simulink model "ZT_VehCtrl_18B_CAN"  (R2018b)
settings: Solver=FixedStepAuto  StartTime=0.0  StopTime=inf  FixedStep=0.005  RelTol=1e-3
InitFcn:
  | mbd_mpc_consistency_checks(bdroot(gcs));
values from neighbouring files (symbols this model uses):
  BatoverTempTh = single(80)    [VCU_INIT.m]
  BRS_PwrValid = single(5)    [VCU_INIT.m]
  BRSEnSpdTh1 = single(10)    [VCU_INIT.m]
  BRSEnSpdTh2 = single(20)    [VCU_INIT.m]
  MCUTempAlarmTh = single (60)    [VCU_INIT.m]
  mps2kmh = single(3.6)    [VCU_INIT.m]
  MtrPwrFac = single(1/9550)    [VCU_INIT.m]
  MtrTempAlarmTh = single (50)    [VCU_INIT.m]
  Padle1Signal1_Th = [PadleSignal1_min,PadleSignal1_max]    [VCU_INIT.m]
  Padle1Signal2_Th = [PadleSignal2_min,PadleSignal2_max]    [VCU_INIT.m]
  PadleSignal1_max = 3.84    [VCU_INIT.m]
  PadleSignal1_min = 0.75    [VCU_INIT.m]
  PadleSignal2_max = 1.92    [VCU_INIT.m]
  PadleSignal2_min = 0.375    [VCU_INIT.m]
  PadleValid = 0.05    [VCU_INIT.m]
  PwrLimFactor = single(0.5)    [VCU_INIT.m]
  Ratio = single(1)    [VCU_INIT.m]
  rpm2mps = single(2*pi/60 * WhlRadius/Ratio)    [VCU_INIT.m]
  SOCLowTh = single(20)    [VCU_INIT.m]
  VehPwrBackwardMax = VehPwrMax * single(0.3)    [VCU_INIT.m]
  VehPwrMax = single(MtrPwrMax * 4)    [VCU_INIT.m]
  VehTrqBackwardMax = VehTrqMax * single(0.3)    [VCU_INIT.m]
  VehTrqMax = single(MtrTrqMax * Ratio *4)    [VCU_INIT.m]
  WhlRadius = single(1)    [VCU_INIT.m]
undefined symbols (not defined in the file or in its folder): Delay_Charge, Delay_Discharge, fifo_0_vect, fifo_1_vect, LQFP, pts1_fifo_0_vect, pts1_fifo_1_vect, pts2_fifo_0_vect, pts2_fifo_1_vect, pts3_fifo_0_vect, pts3_fifo_1_vect, pts4_fifo_0_vect, pts4_fifo_1_vect
libraries: mbd_mpc574x_ec_toolbox x157, canmsglib x74, simulink x38
(part 11 of 12)

== system ZT_VehCtrl_18B_CAN/SigIn/CAN1/TM MCU STATUS 1/UNPACK ==
  ID : Inport
  data : Inport  Port=2
  length : Inport  Port=3
  timestamp : Inport  Port=4
  Action Port : ActionPort  ActionType=case
  Add : Sum
  Bus Creator : BusCreator  Inputs=7  OutDataTypeStr=Bus: CAN_MESSAGE_BUS  NonVirtualBus=on
  Bus Creator1 : BusCreator  Inputs=7
  CAN Unpack6 : canmsglib/CAN Unpack  CANdbFile=D:\VCU\VCU_SL_ZhengZhou\ZT2\模型与接口\CAN_DBC\动力CANB_GBK.dbc  MsgList=(none)  MsgName=TM_MCU_STATUS_1  MsgIDType=Extended (29-bit identifier)  MsgIdentifier=218038277  MsgLength=8  SignalInfo=Active_Discharge_Enable_Feedback$53$1$1$2$1$0$1$0$-Inf$Inf$#IGBT_Enable_Feedback$54$1$1$2$1$0$1$0$-Inf$Inf$#Life_counter$60$4$1$2$1$0$1$0$-Inf$Inf$#Motor_AC_Current$32$16$1$2$1$0$1.000000e-01$0$0$1000$#Motor_Speed$0$16$1$2$1$0$1$-15000$-15000$15000$#Motor_Torque$16$16$1$2$1$0$1$-5000$-5000$5000$#Precharge_Allow$52$1$1$2$1$0$1$0$-Inf$Inf$#  NSignals=7  IDPort=off  TimestampPort=off  ErrorPort=off  RemotePort=off  LengthPort=off  StatusPort=off  StartBits=str2num('[int32(53);int32(54);int32(60);int32(32);int32(0);int32(16);int32(52)]')  SignalSizes=str2num('[int32(1);int32(1);int32(4);int32(16);int32(16);int32(16);int32(1)]')  ByteOrders=str2num('[int32(1);int32(1);int32(1);int32(1);int32(1);int32(1);int32(1)]')  DataTypes=str2num('[int32(2);int32(2);int32(2);int32(2);int32(2);int32(2);int32(2)]')  MultiplexTypes=str2num('[int32(1);int32(1);int32(1);int32(1);int32(1);int32(1);int32(1)]')  MultiplexValues=str2num('[double(0);double(0);double(0);double(0);double(0);double(0);double(0)]')  Factors=str2num('[double(1);double(1);double(1);double(1.000000e-01);double(1);double(1);double(1)]')  Offsets=str2num('[double(0);double(0);double(0);double(0);double(-15000);double(-5000);double(0)]')  Minimums=str2num('[double(-Inf);double(-Inf);double(-Inf);double(0);double(-15000);double(-5000);double(-Inf)]')  Maximums=str2num('[double(Inf);double(Inf);double(Inf);double(1000);double(15000);double(5000);double(Inf)]')  ApplyMinMax=off
      settings: SourceProductName=Simulink Real-Time  SourceProductBaseCode=XP  DataFormat=CANdb specified signals
  Constant : Constant  OutDataTypeStr=uint8
  Constant1 : Constant  OutDataTypeStr=uint8
  Constant4 : Constant  Value=0  OutDataTypeStr=uint8
  Constant5 : Constant  Value=0  OutDataTypeStr=uint8
  Data Store Read : DataStoreRead  DataStoreName=Cnt_TW1
  Data Store Write : DataStoreWrite  DataStoreName=Cnt_TW1
  Data Type Conversion{,14..15,17} (4 alike) : DataTypeConversion  OutDataTypeStr=uint8
  Data Type Conversion1 : DataTypeConversion  OutDataTypeStr=boolean
  Data Type Conversion18 : DataTypeConversion  OutDataTypeStr=uint32
  Data Type Conversion19 : DataTypeConversion  OutDataTypeStr=double
  Data Type Conversion2 : DataTypeConversion  OutDataTypeStr=boolean
  Data Type Conversion{3..6} (4 alike) : DataTypeConversion  OutDataTypeStr=single
  Data Type Conversion7 : DataTypeConversion  OutDataTypeStr=boolean
  Message : Outport
  wires:
  Bus Creator1/1 -> Message/1
  Data Type Conversion15/1 -> Bus Creator/3  "Remote"
  Data Type Conversion14/1 -> Bus Creator/2  "Length"
  Data Type Conversion/1 -> Bus Creator/1  "Extended"
  Bus Creator/1 -> CAN Unpack6/1  "CAN_Msg_In"
  Data Type Conversion17/1 -> Bus Creator/4  "Error"
  timestamp/1 -> Data Type Conversion19/1
  Data Type Conversion19/1 -> Bus Creator/6  "Timestamp"
  ID/1 -> Data Type Conversion18/1
  Constant5/1 -> Data Type Conversion17/1
  Constant1/1 -> Data Type Conversion/1
  Data Type Conversion18/1 -> Bus Creator/5  "ID"
  data/1 -> Bus Creator/7  "Data"
  length/1 -> Data Type Conversion14/1
  Constant4/1 -> Data Type Conversion15/1
  CAN Unpack6/1 -> Data Type Conversion1/1
  CAN Unpack6/2 -> Data Type Conversion2/1
  CAN Unpack6/3 -> Data Type Conversion3/1
  CAN Unpack6/4 -> Data Type Conversion4/1
  CAN Unpack6/5 -> Data Type Conversion5/1
  CAN Unpack6/6 -> Data Type Conversion6/1
  CAN Unpack6/7 -> Data Type Conversion7/1
  Data Type Conversion1/1 -> Bus Creator1/1  "Active_Discharge_Enable_Feedback"
  Data Type Conversion2/1 -> Bus Creator1/2  "IGBT_Enable_Feedback"
  Data Type Conversion3/1 -> Bus Creator1/3  "Life_counter"
  Data Type Conversion4/1 -> Bus Creator1/4  "Motor_AC_Current"
  Data Type Conversion5/1 -> Bus Creator1/5  "Motor_Speed"
  Data Type Conversion6/1 -> Bus Creator1/6  "Motor_Torque"
  Data Type Conversion7/1 -> Bus Creator1/7  "Precharge_Allow"
  Constant/1 -> Add/2
  Data Store Read/1 -> Add/1
  Add/1 -> Data Store Write/1

== system ZT_VehCtrl_18B_CAN/SigIn/CAN1/TM MCU STATUS 2/UNPACK ==
  ID : Inport
  data : Inport  Port=2
  length : Inport  Port=3
  timestamp : Inport  Port=4
  Action Port : ActionPort  ActionType=case
  Add : Sum
  Bus Creator : BusCreator  Inputs=7  OutDataTypeStr=Bus: CAN_MESSAGE_BUS  NonVirtualBus=on
  Bus Creator1 : BusCreator  Inputs=6
  CAN Unpack6 : canmsglib/CAN Unpack  CANdbFile=D:\VCU\VCU_SL_ZhengZhou\ZT2\Module\CAN_DBC\动力CANB_GBK.dbc  MsgList=(none)  MsgName=TM_MCU_STATUS2  MsgIDType=Extended (29-bit identifier)  MsgIdentifier=218038533  MsgLength=8  SignalInfo=Fail_Grade$48$4$1$2$1$0$1$0$-Inf$Inf$#Life_counter$60$4$1$2$1$0$1$0$-Inf$Inf$#MCU_temperature$8$8$1$2$1$0$1$-40$-40$215$#Motor_Temperature$0$8$1$2$1$0$1$-40$-40$215$#Torque_Limit_High$16$16$1$2$1$0$1$0$0$5000$#Torque_Limit_Low$32$16$1$2$1$0$1$-5000$-5000$0$#  NSignals=6  IDPort=off  TimestampPort=off  ErrorPort=off  RemotePort=off  LengthPort=off  StatusPort=off  StartBits=str2num('[int32(48);int32(60);int32(8);int32(0);int32(16);int32(32)]')  SignalSizes=str2num('[int32(4);int32(4);int32(8);int32(8);int32(16);int32(16)]')  ByteOrders=str2num('[int32(1);int32(1);int32(1);int32(1);int32(1);int32(1)]')  DataTypes=str2num('[int32(2);int32(2);int32(2);int32(2);int32(2);int32(2)]')  MultiplexTypes=str2num('[int32(1);int32(1);int32(1);int32(1);int32(1);int32(1)]')  MultiplexValues=str2num('[double(0);double(0);double(0);double(0);double(0);double(0)]')  Factors=str2num('[double(1);double(1);double(1);double(1);double(1);double(1)]')  Offsets=str2num('[double(0);double(0);double(-40);double(-40);double(0);double(-5000)]')  Minimums=str2num('[double(-Inf);double(-Inf);double(-40);double(-40);double(0);double(-5000)]')  Maximums=str2num('[double(Inf);double(Inf);double(215);double(215);double(5000);double(0)]')  ApplyMinMax=off
      settings: SourceProductName=Simulink Real-Time  SourceProductBaseCode=XP  DataFormat=CANdb specified signals
  Constant : Constant  OutDataTypeStr=uint8
  Constant1 : Constant  OutDataTypeStr=uint8
  Constant4 : Constant  Value=0  OutDataTypeStr=uint8
  Constant5 : Constant  Value=0  OutDataTypeStr=uint8
  Data Store Read : DataStoreRead  DataStoreName=Cnt_TW2
  Data Store Write : DataStoreWrite  DataStoreName=Cnt_TW2
  Data Type Conversion{,14..15,17} (4 alike) : DataTypeConversion  OutDataTypeStr=uint8
  Data Type Conversion{1..6} (6 alike) : DataTypeConversion  OutDataTypeStr=single
  Data Type Conversion18 : DataTypeConversion  OutDataTypeStr=uint32
  Data Type Conversion19 : DataTypeConversion  OutDataTypeStr=double
  Message : Outport
  wires:
  Constant4/1 -> Data Type Conversion15/1
  length/1 -> Data Type Conversion14/1
  data/1 -> Bus Creator/7  "Data"
  Data Type Conversion18/1 -> Bus Creator/5  "ID"
  Constant1/1 -> Data Type Conversion/1
  Constant5/1 -> Data Type Conversion17/1
  ID/1 -> Data Type Conversion18/1
  Data Type Conversion19/1 -> Bus Creator/6  "Timestamp"
  timestamp/1 -> Data Type Conversion19/1
  Data Type Conversion17/1 -> Bus Creator/4  "Error"
  Bus Creator/1 -> CAN Unpack6/1  "CAN_Msg_In"
  Data Type Conversion/1 -> Bus Creator/1  "Extended"
  Data Type Conversion14/1 -> Bus Creator/2  "Length"
  Data Type Conversion15/1 -> Bus Creator/3  "Remote"
  Bus Creator1/1 -> Message/1
  CAN Unpack6/4 -> Data Type Conversion4/1
  CAN Unpack6/3 -> Data Type Conversion3/1
  CAN Unpack6/5 -> Data Type Conversion5/1
  CAN Unpack6/2 -> Data Type Conversion2/1
  CAN Unpack6/6 -> Data Type Conversion6/1
  CAN Unpack6/1 -> Data Type Conversion1/1
  Data Type Conversion1/1 -> Bus Creator1/1  "Fail_Grade"
  Data Type Conversion2/1 -> Bus Creator1/2  "Life_counter"
  Data Type Conversion3/1 -> Bus Creator1/3  "MCU_temperature"
  Data Type Conversion4/1 -> Bus Creator1/4  "Motor_Temperature"
  Data Type Conversion5/1 -> Bus Creator1/5  "Torque_Limit_High"
  Data Type Conversion6/1 -> Bus Creator1/6  "Torque_Limit_Low"
  Constant/1 -> Add/2
  Add/1 -> Data Store Write/1
  Data Store Read/1 -> Add/1

== system ZT_VehCtrl_18B_CAN/SigIn/CAN1/TM MCU STATUS 3/UNPACK ==
  ID : Inport
  data : Inport  Port=2
  length : Inport  Port=3
  timestamp : Inport  Port=4
  Action Port : ActionPort  ActionType=case
  Add : Sum
  Bus Creator : BusCreator  Inputs=7  OutDataTypeStr=Bus: CAN_MESSAGE_BUS  NonVirtualBus=on
  Bus Creator1 : BusCreator  Inputs=5
  CAN Unpack6 : canmsglib/CAN Unpack  CANdbFile=D:\VCU\VCU_SL_ZhengZhou\ZT2\Module\CAN_DBC\动力CANB_GBK.dbc  MsgList=(none)  MsgName=TM_MCU_STATUS3  MsgIDType=Extended (29-bit identifier)  MsgIdentifier=218038789  MsgLength=8  SignalInfo=Alarm_Code$8$8$1$2$1$0$1$0$0$255$#DC_Current_A$16$16$1$2$1$0$1$-1000$-1000$1000$#DC_Voltage_V$32$16$1$2$1$0$1.000000e-01$0$0$1000$#Fault_Code$0$8$1$2$1$0$1$0$0$255$#Life_counter$48$4$1$2$1$0$1$0$0$15$#  NSignals=5  IDPort=off  TimestampPort=off  ErrorPort=off  RemotePort=off  LengthPort=off  StatusPort=off  StartBits=str2num('[int32(8);int32(16);int32(32);int32(0);int32(48)]')  SignalSizes=str2num('[int32(8);int32(16);int32(16);int32(8);int32(4)]')  ByteOrders=str2num('[int32(1);int32(1);int32(1);int32(1);int32(1)]')  DataTypes=str2num('[int32(2);int32(2);int32(2);int32(2);int32(2)]')  MultiplexTypes=str2num('[int32(1);int32(1);int32(1);int32(1);int32(1)]')  MultiplexValues=str2num('[double(0);double(0);double(0);double(0);double(0)]')  Factors=str2num('[double(1);double(1);double(1.000000e-01);double(1);double(1)]')  Offsets=str2num('[double(0);double(-1000);double(0);double(0);double(0)]')  Minimums=str2num('[double(0);double(-1000);double(0);double(0);double(0)]')  Maximums=str2num('[double(255);double(1000);double(1000);double(255);double(15)]')  ApplyMinMax=off
      settings: SourceProductName=Simulink Real-Time  SourceProductBaseCode=XP  DataFormat=CANdb specified signals
  Constant : Constant  OutDataTypeStr=uint8
  Constant1 : Constant  OutDataTypeStr=uint8
  Constant4 : Constant  Value=0  OutDataTypeStr=uint8
  Constant5 : Constant  Value=0  OutDataTypeStr=uint8
  Data Store Read : DataStoreRead  DataStoreName=Cnt_TW3
  Data Store Write : DataStoreWrite  DataStoreName=Cnt_TW3
  Data Type Conversion{,14..15,17} (4 alike) : DataTypeConversion  OutDataTypeStr=uint8
  Data Type Conversion{1..5} (5 alike) : DataTypeConversion  OutDataTypeStr=single
  Data Type Conversion18 : DataTypeConversion  OutDataTypeStr=uint32
  Data Type Conversion19 : DataTypeConversion  OutDataTypeStr=double
  Message : Outport
  wires:
  Bus Creator1/1 -> Message/1
  Data Type Conversion15/1 -> Bus Creator/3  "Remote"
  Data Type Conversion14/1 -> Bus Creator/2  "Length"
  Data Type Conversion/1 -> Bus Creator/1  "Extended"
  Bus Creator/1 -> CAN Unpack6/1  "CAN_Msg_In"
  Data Type Conversion17/1 -> Bus Creator/4  "Error"
  timestamp/1 -> Data Type Conversion19/1
  Data Type Conversion19/1 -> Bus Creator/6  "Timestamp"
  ID/1 -> Data Type Conversion18/1
  Constant5/1 -> Data Type Conversion17/1
  Constant1/1 -> Data Type Conversion/1
  Data Type Conversion18/1 -> Bus Creator/5  "ID"
  data/1 -> Bus Creator/7  "Data"
  length/1 -> Data Type Conversion14/1
  Constant4/1 -> Data Type Conversion15/1
  CAN Unpack6/1 -> Data Type Conversion1/1
  CAN Unpack6/2 -> Data Type Conversion2/1
  CAN Unpack6/3 -> Data Type Conversion3/1
  CAN Unpack6/4 -> Data Type Conversion4/1
  CAN Unpack6/5 -> Data Type Conversion5/1
  Data Type Conversion1/1 -> Bus Creator1/1  "Alarm_Code"
  Data Type Conversion2/1 -> Bus Creator1/2  "DC_Current_A"
  Data Type Conversion3/1 -> Bus Creator1/3  "DC_Voltage_A"
  Data Type Conversion4/1 -> Bus Creator1/4  "Fault_Code"
  Data Type Conversion5/1 -> Bus Creator1/5  "Life_counter"
  Constant/1 -> Add/2
  Add/1 -> Data Store Write/1
  Data Store Read/1 -> Add/1

== system ZT_VehCtrl_18B_CAN/SigIn/CAN1/TWV /UNPACK ==
  ID : Inport
  data : Inport  Port=2
  length : Inport  Port=3
  timestamp : Inport  Port=4
  Action Port : ActionPort  ActionType=case
  Add : Sum
  Bus Creator : BusCreator  Inputs=7  OutDataTypeStr=Bus: CAN_MESSAGE_BUS  NonVirtualBus=on
  Bus Creator1 : BusCreator  Inputs=9
  CAN Unpack6 : canmsglib/CAN Unpack  CANdbFile=D:\VCU\VCU_SL_ZhengZhou\ZT2\模型与接口\CAN_DBC\动力CANB_GBK.dbc  MsgList=(none)  MsgName=TWV  MsgIDType=Extended (29-bit identifier)  MsgIdentifier=419374139  MsgLength=8  SignalInfo=TWV1_P_MotorOpenCircuitFlt$6$1$1$2$1$0$1$0$0$1$#TWV1_P_MotorSta$7$1$1$2$1$0$1$0$0$1$#TWV1_P_OverCurrent$2$1$1$2$1$0$1$0$0$1$#TWV1_P_OverTempFlt$3$1$1$2$1$0$1$0$0$1$#TWV1_P_OverVoltageFlt$1$1$1$2$1$0$1$0$0$1$#TWV1_P_RESP_ERROR$0$1$1$2$1$0$1$0$0$1$#TWV1_P_RealSta$8$8$1$2$1$0$4.000000e-01$0$0$100$#TWV1_P_StallFlt$5$1$1$2$1$0$1$0$0$1$#TWV1_P_UnderVoltageFlt$4$1$1$2$1$0$1$0$0$1$#  NSignals=9  IDPort=off  TimestampPort=off  ErrorPort=off  RemotePort=off  LengthPort=off  StatusPort=off  StartBits=str2num('[int32(6);int32(7);int32(2);int32(3);int32(1);int32(0);int32(8);int32(5);int32(4)]')  SignalSizes=str2num('[int32(1);int32(1);int32(1);int32(1);int32(1);int32(1);int32(8);int32(1);int32(1)]')  ByteOrders=str2num('[int32(1);int32(1);int32(1);int32(1);int32(1);int32(1);int32(1);int32(1);int32(1)]')  DataTypes=str2num('[int32(2);int32(2);int32(2);int32(2);int32(2);int32(2);int32(2);int32(2);int32(2)]')  MultiplexTypes=str2num('[int32(1);int32(1);int32(1);int32(1);int32(1);int32(1);int32(1);int32(1);int32(1)]')  MultiplexValues=str2num('[double(0);double(0);double(0);double(0);double(0);double(0);double(0);double(0);double(0)]')  Factors=str2num('[double(1);double(1);double(1);double(1);double(1);double(1);double(4.000000e-01);double(1);double(1)]')  Offsets=str2num('[double(0);double(0);double(0);double(0);double(0);double(0);double(0);double(0);double(0)]')  Minimums=str2num('[double(0);double(0);double(0);double(0);double(0);double(0);double(0);double(0);double(0)]')  Maximums=str2num('[double(1);double(1);double(1);double(1);double(1);double(1);double(100);double(1);double(1)]')  ApplyMinMax=off
      settings: SourceProductName=Simulink Real-Time  SourceProductBaseCode=XP  DataFormat=CANdb specified signals
  Constant : Constant  OutDataTypeStr=uint8
  Constant1 : Constant  OutDataTypeStr=uint8
  Constant4 : Constant  Value=0  OutDataTypeStr=uint8
  Constant5 : Constant  Value=0  OutDataTypeStr=uint8
  Data Store Read : DataStoreRead  DataStoreName=Cnt_TWV
  Data Store Write : DataStoreWrite  DataStoreName=Cnt_TWV
  Data Type Conversion{,14..15,17} (4 alike) : DataTypeConversion  OutDataTypeStr=uint8
  Data Type Conversion{1..6,8..9} (8 alike) : DataTypeConversion  OutDataTypeStr=boolean
  Data Type Conversion18 : DataTypeConversion  OutDataTypeStr=uint32
  Data Type Conversion19 : DataTypeConversion  OutDataTypeStr=double
  Data Type Conversion7 : DataTypeConversion  OutDataTypeStr=single
  Message : Outport
  wires:
  Constant4/1 -> Data Type Conversion15/1
  length/1 -> Data Type Conversion14/1
  data/1 -> Bus Creator/7  "Data"
  Data Type Conversion18/1 -> Bus Creator/5  "ID"
  Constant1/1 -> Data Type Conversion/1
  Constant5/1 -> Data Type Conversion17/1
  ID/1 -> Data Type Conversion18/1
  Data Type Conversion19/1 -> Bus Creator/6  "Timestamp"
  timestamp/1 -> Data Type Conversion19/1
  Data Type Conversion17/1 -> Bus Creator/4  "Error"
  Bus Creator/1 -> CAN Unpack6/1  "CAN_Msg_In"
  Data Type Conversion/1 -> Bus Creator/1  "Extended"
  Data Type Conversion14/1 -> Bus Creator/2  "Length"
  Data Type Conversion15/1 -> Bus Creator/3  "Remote"
  Bus Creator1/1 -> Message/1
  CAN Unpack6/1 -> Data Type Conversion1/1
  CAN Unpack6/2 -> Data Type Conversion2/1
  CAN Unpack6/3 -> Data Type Conversion3/1
  CAN Unpack6/4 -> Data Type Conversion4/1
  CAN Unpack6/5 -> Data Type Conversion5/1
  CAN Unpack6/6 -> Data Type Conversion6/1
  CAN Unpack6/7 -> Data Type Conversion7/1
  CAN Unpack6/8 -> Data Type Conversion8/1
  CAN Unpack6/9 -> Data Type Conversion9/1
  Data Type Conversion1/1 -> Bus Creator1/1  "TWV1_P_MotorOpenCircuitFlt"
  Data Type Conversion2/1 -> Bus Creator1/2  "TWV1_P_MotorSta"
  Data Type Conversion3/1 -> Bus Creator1/3  "TWV1_P_OverCurrent"
  Data Type Conversion4/1 -> Bus Creator1/4  "TWV1_P_OverTempFlt"
  Data Type Conversion5/1 -> Bus Creator1/5  "TWV1_P_OverVoltageFlt"
  Data Type Conversion6/1 -> Bus Creator1/6  "TWV1_P_RESP_ERROR"
  Data Type Conversion7/1 -> Bus Creator1/7  "TWV1_P_RealSta"
  Data Type Conversion8/1 -> Bus Creator1/8  "TWV1_P_StallFlt"
  Data Type Conversion9/1 -> Bus Creator1/9  "TWV1_P_UnderVoltageFlt"
  Constant/1 -> Add/2
  Data Store Read/1 -> Add/1
  Add/1 -> Data Store Write/1

== system ZT_VehCtrl_18B_CAN/SigIn/PWM/PWM_PTS1/Subsystem ==
  In1 : Inport
  Add2 : Sum  AccumDataTypeStr=single
  Constant : Constant  OutDataTypeStr=uint8
  Constant1 : Constant  Value=0  OutDataTypeStr=single
  Data Store Read3 : DataStoreRead  DataStoreName=pts1_pwm_cnt
  Data Store Write : DataStoreWrite  DataStoreName=pts1_pwm_cnt
  Saturation : Saturate  UpperLimit=100  LowerLimit=0
  Switch : Switch  Criteria=u2 > Threshold  Threshold=100
  Out1 : Outport  VectorParamsAs1DForOutWhenUnconnected=on
  wires:
  Saturation/1 -> Data Store Write/1
  Add2/1 -> Switch/2, Saturation/1
  Data Store Read3/1 -> Add2/2
  Constant1/1 -> Switch/1
  Switch/1 -> Out1/1
  Constant/1 -> Add2/1
  In1/1 -> Switch/3

== system ZT_VehCtrl_18B_CAN/SigIn/PWM/PWM_PTS1/Subsystem_capture ==
  In1 : Inport
  function : TriggerPort  TriggerType=function-call  VariantControl=Variant
  Constant : Constant  Value=0  OutDataTypeStr=uint8
  Counter Limited : simulink/Sources/Counter Limited  uplimit=7  tsamp=-1
  Data Store Write : DataStoreWrite  DataStoreName=pts1_pwm_cnt
  Data Store Write3 : DataStoreWrite  DataStoreName=pwm3_cnt
  Terminator : Terminator
  eTimer_Arm_Capture : mbd_mpc574x_ec_toolbox/Motor Control Blocks/eTIMER Blocks/eTimer_Arm_Capture  etimerModule=1  etimerChannel=2  etimerArmAction=Stop
  eTimer_Capture : mbd_mpc574x_ec_toolbox/Motor Control Blocks/eTIMER Blocks/eTimer_Capture  etimerModule=1  etimerChannel=2
      settings: SourceProductName=NXP Model-Based Design Toolbox for MPC57xx MCUs
  Out1 : Outport  OutDataTypeStr=uint16
  Out2 : Outport  Port=2  OutDataTypeStr=uint16
  Out3 : Outport  Port=3  OutDataTypeStr=uint16
  Out4 : Outport  Port=4  OutDataTypeStr=uint16
  wires:
  eTimer_Capture/1 -> Out1/1
  eTimer_Capture/4 -> Out4/1
  eTimer_Capture/3 -> Out3/1
  eTimer_Capture/2 -> Out2/1
  In1/1 -> Terminator/1
  Constant/1 -> Data Store Write/1
  Counter Limited/1 -> Data Store Write3/1

== system ZT_VehCtrl_18B_CAN/SigIn/PWM/PWM_PTS2/Subsystem ==
  In1 : Inport
  Add2 : Sum  AccumDataTypeStr=single
  Constant : Constant  OutDataTypeStr=uint8
  Constant1 : Constant  Value=0  OutDataTypeStr=single
  Data Store Read3 : DataStoreRead  DataStoreName=pts2_pwm_cnt
  Data Store Write : DataStoreWrite  DataStoreName=pts2_pwm_cnt
  Saturation : Saturate  UpperLimit=100  LowerLimit=0
  Switch : Switch  Criteria=u2 > Threshold  Threshold=100
  Out1 : Outport  VectorParamsAs1DForOutWhenUnconnected=on
  wires:
  In1/1 -> Switch/3
  Constant/1 -> Add2/1
  Switch/1 -> Out1/1
  Constant1/1 -> Switch/1
  Data Store Read3/1 -> Add2/2
  Add2/1 -> Saturation/1, Switch/2
  Saturation/1 -> Data Store Write/1

== system ZT_VehCtrl_18B_CAN/SigIn/PWM/PWM_PTS2/Subsystem_capture ==
  In1 : Inport
  function : TriggerPort  TriggerType=function-call  VariantControl=Variant
  Constant : Constant  Value=0  OutDataTypeStr=uint8
  Counter Limited : simulink/Sources/Counter Limited  uplimit=255  tsamp=-1
  Data Store Write : DataStoreWrite  DataStoreName=pts2_pwm_cnt
  Data Store Write2 : DataStoreWrite  DataStoreName=pwm2_cnt
  Terminator : Terminator
  eTimer_Arm_Capture : mbd_mpc574x_ec_toolbox/Motor Control Blocks/eTIMER Blocks/eTimer_Arm_Capture  etimerModule=1  etimerChannel=3  etimerArmAction=Stop
  eTimer_Capture : mbd_mpc574x_ec_toolbox/Motor Control Blocks/eTIMER Blocks/eTimer_Capture  etimerModule=1  etimerChannel=3
      settings: SourceProductName=NXP Model-Based Design Toolbox for MPC57xx MCUs
  Out1 : Outport  OutDataTypeStr=uint16
  Out2 : Outport  Port=2  OutDataTypeStr=uint16
  Out3 : Outport  Port=3  OutDataTypeStr=uint16
  Out4 : Outport  Port=4  OutDataTypeStr=uint16
  wires:
  Constant/1 -> Data Store Write/1
  In1/1 -> Terminator/1
  eTimer_Capture/2 -> Out2/1
  eTimer_Capture/3 -> Out3/1
  eTimer_Capture/4 -> Out4/1
  eTimer_Capture/1 -> Out1/1
  Counter Limited/1 -> Data Store Write2/1

== system ZT_VehCtrl_18B_CAN/SigIn/PWM/PWM_PTS3/Subsystem ==
  In1 : Inport
  Add2 : Sum  AccumDataTypeStr=single
  Constant : Constant  OutDataTypeStr=uint8
  Constant1 : Constant  Value=0  OutDataTypeStr=single
  Data Store Read3 : DataStoreRead  DataStoreName=pts3_pwm_cnt
  Data Store Write : DataStoreWrite  DataStoreName=pts3_pwm_cnt
  Saturation : Saturate  UpperLimit=100  LowerLimit=0
  Switch : Switch  Criteria=u2 > Threshold  Threshold=100
  Out1 : Outport  VectorParamsAs1DForOutWhenUnconnected=on
  wires:
  Saturation/1 -> Data Store Write/1
  Add2/1 -> Switch/2, Saturation/1
  Data Store Read3/1 -> Add2/2
  Constant1/1 -> Switch/1
  Switch/1 -> Out1/1
  Constant/1 -> Add2/1
  In1/1 -> Switch/3

== system ZT_VehCtrl_18B_CAN/SigIn/PWM/PWM_PTS3/Subsystem_capture ==
  In1 : Inport
  function : TriggerPort  TriggerType=function-call  VariantControl=Variant
  Constant : Constant  Value=0  OutDataTypeStr=uint8
  Counter Limited : simulink/Sources/Counter Limited  uplimit=255  tsamp=-1
  Data Store Write : DataStoreWrite  DataStoreName=pts3_pwm_cnt
  Data Store Write4 : DataStoreWrite  DataStoreName=pwm4_cnt
  Terminator : Terminator
  eTimer_Arm_Capture : mbd_mpc574x_ec_toolbox/Motor Control Blocks/eTIMER Blocks/eTimer_Arm_Capture  etimerModule=1  etimerChannel=1  etimerArmAction=Stop
  eTimer_Capture : mbd_mpc574x_ec_toolbox/Motor Control Blocks/eTIMER Blocks/eTimer_Capture  etimerModule=1  etimerChannel=1
      settings: SourceProductName=NXP Model-Based Design Toolbox for MPC57xx MCUs
  Out1 : Outport  OutDataTypeStr=uint16
  Out2 : Outport  Port=2  OutDataTypeStr=uint16
  Out3 : Outport  Port=3  OutDataTypeStr=uint16
  Out4 : Outport  Port=4  OutDataTypeStr=uint16
  wires:
  eTimer_Capture/1 -> Out1/1
  eTimer_Capture/4 -> Out4/1
  eTimer_Capture/3 -> Out3/1
  eTimer_Capture/2 -> Out2/1
  In1/1 -> Terminator/1
  Constant/1 -> Data Store Write/1
  Counter Limited/1 -> Data Store Write4/1

== system ZT_VehCtrl_18B_CAN/SigIn/PWM/PWM_PTS4/Subsystem ==
  In1 : Inport
  Add2 : Sum  AccumDataTypeStr=single
  Constant : Constant  OutDataTypeStr=uint8
  Constant1 : Constant  Value=0  OutDataTypeStr=single
  Data Store Read3 : DataStoreRead  DataStoreName=pts4_pwm_cnt
  Data Store Write : DataStoreWrite  DataStoreName=pts4_pwm_cnt
  Saturation : Saturate  UpperLimit=100  LowerLimit=0
  Switch : Switch  Criteria=u2 > Threshold  Threshold=100
  Out1 : Outport  VectorParamsAs1DForOutWhenUnconnected=on
  wires:
  In1/1 -> Switch/3
  Constant/1 -> Add2/1
  Switch/1 -> Out1/1
  Constant1/1 -> Switch/1
  Data Store Read3/1 -> Add2/2
  Add2/1 -> Saturation/1, Switch/2
  Saturation/1 -> Data Store Write/1

== system ZT_VehCtrl_18B_CAN/SigIn/PWM/PWM_PTS4/Subsystem_capture ==
  In1 : Inport
  function : TriggerPort  TriggerType=function-call  VariantControl=Variant
  Constant : Constant  Value=0  OutDataTypeStr=uint8
  Counter Limited : simulink/Sources/Counter Limited  uplimit=255  tsamp=-1
  Data Store Write : DataStoreWrite  DataStoreName=pts4_pwm_cnt
  Data Store Write1 : DataStoreWrite  DataStoreName=pwm1_cnt
  Terminator : Terminator
  eTimer_Arm_Capture : mbd_mpc574x_ec_toolbox/Motor Control Blocks/eTIMER Blocks/eTimer_Arm_Capture  etimerModule=0  etimerChannel=2  etimerArmAction=Stop
  eTimer_Capture : mbd_mpc574x_ec_toolbox/Motor Control Blocks/eTIMER Blocks/eTimer_Capture  etimerModule=0  etimerChannel=2
      settings: SourceProductName=NXP Model-Based Design Toolbox for MPC57xx MCUs
  Out1 : Outport  OutDataTypeStr=uint16
  Out2 : Outport  Port=2  OutDataTypeStr=uint16
  Out3 : Outport  Port=3  OutDataTypeStr=uint16
  Out4 : Outport  Port=4  OutDataTypeStr=uint16
  wires:
  Constant/1 -> Data Store Write/1
  In1/1 -> Terminator/1
  eTimer_Capture/2 -> Out2/1
  eTimer_Capture/3 -> Out3/1
  eTimer_Capture/4 -> Out4/1
  eTimer_Capture/1 -> Out1/1
  Counter Limited/1 -> Data Store Write1/1

== system ZT_VehCtrl_18B_CAN/SigIn/PWM/Subsystem/Frequency_DutyCycle_Computation ==
  Add : Sum  Inputs=+-  AccumDataTypeStr=single
  Add1 : Sum  Inputs=+-  AccumDataTypeStr=single
  Data Store Read : DataStoreRead  DataStoreName=fifo_0_vect  DataStoreElements=fifo_0_vect(2)#fifo_0_vect(1)
  Data Store Read1 : DataStoreRead  DataStoreName=fifo_1_vect  DataStoreElements=fifo_1_vect(1)
  Data Store Read2 : DataStoreRead  DataStoreName=fifo_0_vect  DataStoreElements=fifo_0_vect(1)
  Divide : Product  Inputs=*/  OutDataTypeStr=single
  Divide1 : Product  Inputs=*//
  Freq_MC : Constant  Value=80000000  OutDataTypeStr=single
  Prescaler : Constant  Value=32  OutDataTypeStr=single
  Out1 : Outport
  Out2 : Outport  Port=2
  wires:
  Data Store Read1/1 -> Add1/1
  Data Store Read/2 -> Add/2
  Divide1/1 -> Out2/1
  Add/1 -> Divide/2, Divide1/3
  Add1/1 -> Divide/1
  Divide/1 -> Out1/1
  Data Store Read/1 -> Add/1
  Freq_MC/1 -> Divide1/1
  Prescaler/1 -> Divide1/2
  Data Store Read2/1 -> Add1/2

== system ZT_VehCtrl_18B_CAN/SigIn/PWM/Subsystem/eTimer Configuration and Signal Measurements ==
  Subsystem_capture : Subsystem
  eTimer_Arm_Capture : mbd_mpc574x_ec_toolbox/Motor Control Blocks/eTIMER Blocks/eTimer_Arm_Capture  etimerModule=0  etimerChannel=1  etimerArmAction=Start
  eTimer_Config : mbd_mpc574x_ec_toolbox/Motor Control Blocks/eTIMER Blocks/eTimer_Config  etimerModule=0  etimerChannel=1  etimerMode=COUNT Mode  etimerCountOnce=Count repeatedly  etimerCountLength=Continue counting to roll over  etimerCountDirection=Count up  etimerCountStart=on  etimerCaptureArm=on  etimerShowAdv=on  etimerPrimarySource=IP Bus clock divide by 32 prescaler  etimerPrimaryPolarity=True polarity  etimerSecondarySource=Counter 0 input pin  etimerSecondaryPolarity=True polarity  etimerSampleCount=Require 3 consecutive samples to be of equal value  etimerSamplePeriod=0  etimerOutEnable=The external pin is configured as an input  etimerOutPolarity=True polarity  etimerOutMode=Toggle OFLAG output using alternating compare registers  etimerCompMode="COMP1 and COMP2  are used when the counter is counting up"  etimerCompLoad1=COMP1 is never preload  etimerCompLoad2=COMP2 is never preload  etimerCapt1=Capture rising edges  etimerCapt2=Capture falling edges  etimerOneShot=Free running mode is selected  etimerMasterMode=Disable broadcast of this channel output  etimerCoForce=Other channels cannot force this channel output  etimerCoChanInit=Other channels cannot force re-initialization of this channel  etimerRedundant=off  etimerCOMP1init=0  etimerCOMP2init=0  etimerCNTRinit=0  etimerCh0=PTA0: [eTimer0_ETC0 | eTimer_0 Input Data Channel 0]  etimerCh1=None  etimerCh2=None  etimerCh3=None  etimerCh4=None  etimerCh5=None  etimerIsrTCFIE=off  etimerIsrTCF1IE=off  etimerIsrTCF2IE=off  etimerIsrTOFIE=off  etimerIsrIELFIE=off  etimerIsrIEHFIE=off  etimerIsrICF1IE=off  etimerIsrICF2IE=on  etimerIsrRCF=off  etimerIsrWDF=off
  eTimer_ISR : mbd_mpc574x_ec_toolbox/Motor Control Blocks/eTIMER Blocks/eTimer_ISR_Handler  etimerModule=0  etimerInterrupt=Channel Interrupt  etimerChannel=1  etimerIsrPriority=14
  Out1 : Outport
  Out2 : Outport  Port=2
  Out3 : Outport  Port=3
  Out4 : Outport  Port=4
  wires:
  eTimer_ISR/1 -> Subsystem_capture/Trigger
  eTimer_ISR/2 -> Subsystem_capture/1(In1)
  Subsystem_capture/1(Out1) -> Out1/1
  Subsystem_capture/2(Out2) -> Out2/1
  Subsystem_capture/3(Out3) -> Out3/1
  Subsystem_capture/4(Out4) -> Out4/1

== system ZT_VehCtrl_18B_CAN/SigOut/GPIO /ETC/Subsystem ==
  COMPLD1 : Inport
  COMPLD2 : Inport  Port=2
  Constant4 : Constant  Value=0  OutDataTypeStr=Inherit: Inherit via back propagation
  Data Type Conversion : DataTypeConversion
  Data Type Conversion1 : DataTypeConversion
  Data Type Conversion2 : DataTypeConversion
  eTimer_Preload2 : mbd_mpc574x_ec_toolbox/Motor Control Blocks/eTIMER Blocks/eTimer_Preload  etimerModule=0  etimerChannel=3
      settings: SourceProductName=NXP Model-Based Design Toolbox for MPC57xx MCUs
  eTimer_Start_Stop_Timer1 : mbd_mpc574x_ec_toolbox/Motor Control Blocks/eTIMER Blocks/eTimer_Start_Stop_Timer  etimerModule=0  etimerChannel=3  etimerAction=Start
      settings: SourceProductName=NXP Model-Based Design Toolbox for MPC57xx MCUs
  wires:
  Constant4/1 -> Data Type Conversion/1
  COMPLD2/1 -> Data Type Conversion2/1
  COMPLD1/1 -> Data Type Conversion1/1
  Data Type Conversion/1 -> eTimer_Preload2/1
  Data Type Conversion1/1 -> eTimer_Preload2/2
  Data Type Conversion2/1 -> eTimer_Preload2/3

== system ZT_VehCtrl_18B_CAN/SigOut/GPIO /ETC/Subsystem1 ==
  COMPLD1 : Inport
  COMPLD2 : Inport  Port=2
  Constant4 : Constant  Value=0  OutDataTypeStr=Inherit: Inherit via back propagation
  Data Type Conversion : DataTypeConversion
  Data Type Conversion1 : DataTypeConversion
  Data Type Conversion2 : DataTypeConversion
  eTimer_Preload2 : mbd_mpc574x_ec_toolbox/Motor Control Blocks/eTIMER Blocks/eTimer_Preload  etimerModule=2  etimerChannel=2
      settings: SourceProductName=NXP Model-Based Design Toolbox for MPC57xx MCUs
  eTimer_Start_Stop_Timer1 : mbd_mpc574x_ec_toolbox/Motor Control Blocks/eTIMER Blocks/eTimer_Start_Stop_Timer  etimerModule=2  etimerChannel=2  etimerAction=Start
      settings: SourceProductName=NXP Model-Based Design Toolbox for MPC57xx MCUs
  wires:
  COMPLD1/1 -> Data Type Conversion1/1
  COMPLD2/1 -> Data Type Conversion2/1
  Constant4/1 -> Data Type Conversion/1
  Data Type Conversion/1 -> eTimer_Preload2/1
  Data Type Conversion1/1 -> eTimer_Preload2/2
  Data Type Conversion2/1 -> eTimer_Preload2/3

== system ZT_VehCtrl_18B_CAN/SigOut/GPIO /ETC/Subsystem2 ==
  COMPLD1 : Inport
  COMPLD2 : Inport  Port=2
  Constant4 : Constant  Value=0  OutDataTypeStr=Inherit: Inherit via back propagation
  Data Type Conversion : DataTypeConversion
  Data Type Conversion1 : DataTypeConversion
  Data Type Conversion2 : DataTypeConversion
  eTimer_Preload2 : mbd_mpc574x_ec_toolbox/Motor Control Blocks/eTIMER Blocks/eTimer_Preload  etimerModule=0  etimerChannel=5
      settings: SourceProductName=NXP Model-Based Design Toolbox for MPC57xx MCUs
  eTimer_Start_Stop_Timer1 : mbd_mpc574x_ec_toolbox/Motor Control Blocks/eTIMER Blocks/eTimer_Start_Stop_Timer  etimerModule=0  etimerChannel=5  etimerAction=Start
      settings: SourceProductName=NXP Model-Based Design Toolbox for MPC57xx MCUs
  wires:
  Constant4/1 -> Data Type Conversion/1
  COMPLD2/1 -> Data Type Conversion2/1
  COMPLD1/1 -> Data Type Conversion1/1
  Data Type Conversion/1 -> eTimer_Preload2/1
  Data Type Conversion1/1 -> eTimer_Preload2/2
  Data Type Conversion2/1 -> eTimer_Preload2/3

== system ZT_VehCtrl_18B_CAN/SigOut/GPIO /ETC/Subsystem3 ==
  COMPLD1 : Inport
  COMPLD2 : Inport  Port=2
  Constant4 : Constant  Value=0  OutDataTypeStr=Inherit: Inherit via back propagation
  Data Type Conversion : DataTypeConversion
  Data Type Conversion1 : DataTypeConversion
  Data Type Conversion2 : DataTypeConversion
  eTimer_Preload2 : mbd_mpc574x_ec_toolbox/Motor Control Blocks/eTIMER Blocks/eTimer_Preload  etimerModule=1  etimerChannel=4
      settings: SourceProductName=NXP Model-Based Design Toolbox for MPC57xx MCUs
  eTimer_Start_Stop_Timer1 : mbd_mpc574x_ec_toolbox/Motor Control Blocks/eTIMER Blocks/eTimer_Start_Stop_Timer  etimerModule=1  etimerChannel=4  etimerAction=Start
      settings: SourceProductName=NXP Model-Based Design Toolbox for MPC57xx MCUs
  wires:
  Data Type Conversion2/1 -> eTimer_Preload2/3
  Data Type Conversion1/1 -> eTimer_Preload2/2
  Data Type Conversion/1 -> eTimer_Preload2/1
  COMPLD1/1 -> Data Type Conversion1/1
  COMPLD2/1 -> Data Type Conversion2/1
  Constant4/1 -> Data Type Conversion/1

== system ZT_VehCtrl_18B_CAN/SigOut/GPIO /ETC/Subsystem4 ==
  COMPLD1 : Inport
  COMPLD2 : Inport  Port=2
  Constant4 : Constant  Value=0  OutDataTypeStr=Inherit: Inherit via back propagation
  Data Type Conversion : DataTypeConversion
  Data Type Conversion1 : DataTypeConversion
  Data Type Conversion2 : DataTypeConversion
  eTimer_Preload2 : mbd_mpc574x_ec_toolbox/Motor Control Blocks/eTIMER Blocks/eTimer_Preload  etimerModule=1  etimerChannel=5
      settings: SourceProductName=NXP Model-Based Design Toolbox for MPC57xx MCUs
  eTimer_Start_Stop_Timer1 : mbd_mpc574x_ec_toolbox/Motor Control Blocks/eTIMER Blocks/eTimer_Start_Stop_Timer  etimerModule=1  etimerChannel=5  etimerAction=Start
      settings: SourceProductName=NXP Model-Based Design Toolbox for MPC57xx MCUs
  wires:
  Data Type Conversion2/1 -> eTimer_Preload2/3
  Data Type Conversion1/1 -> eTimer_Preload2/2
  Data Type Conversion/1 -> eTimer_Preload2/1
  Constant4/1 -> Data Type Conversion/1
  COMPLD2/1 -> Data Type Conversion2/1
  COMPLD1/1 -> Data Type Conversion1/1

== system ZT_VehCtrl_18B_CAN/SigOut/GPIO /ETC/Subsystem5 ==
  COMPLD1 : Inport
  COMPLD2 : Inport  Port=2
  Constant4 : Constant  Value=0  OutDataTypeStr=Inherit: Inherit via back propagation
  Data Type Conversion : DataTypeConversion
  Data Type Conversion1 : DataTypeConversion
  Data Type Conversion2 : DataTypeConversion
  eTimer_Preload2 : mbd_mpc574x_ec_toolbox/Motor Control Blocks/eTIMER Blocks/eTimer_Preload  etimerModule=1  etimerChannel=0
      settings: SourceProductName=NXP Model-Based Design Toolbox for MPC57xx MCUs
  eTimer_Start_Stop_Timer1 : mbd_mpc574x_ec_toolbox/Motor Control Blocks/eTIMER Blocks/eTimer_Start_Stop_Timer  etimerModule=1  etimerChannel=0  etimerAction=Start
      settings: SourceProductName=NXP Model-Based Design Toolbox for MPC57xx MCUs
  wires:
  Data Type Conversion2/1 -> eTimer_Preload2/3
  Data Type Conversion1/1 -> eTimer_Preload2/2
  Data Type Conversion/1 -> eTimer_Preload2/1
  COMPLD1/1 -> Data Type Conversion1/1
  COMPLD2/1 -> Data Type Conversion2/1
  Constant4/1 -> Data Type Conversion/1

== system ZT_VehCtrl_18B_CAN/SigOut/GPIO /PWM_OUT/PWM Configuration and Frequency Update ==
  In1 : Inport
  In2 : Inport  Port=2
  FlexPWM_Config : mbd_mpc574x_ec_toolbox/Motor Control Blocks/FlexPWM Blocks/FlexPWM_Config  Priority=1  pwmModule=0  pwmSubmodule=3  pwmMode=Edge aligned PWM  pwmPair=Independent  pwmCompSource=PWM23  pwmCounterInit=Local sync (PWMX)  pwmClockSource=Peripheral clock  pwmUnits=Hz  pwmFrequency=10000  pwmPeriod=8000  pwmPrescaler=Divide by 1  pwmDtUnits=Nanoseconds  pwmDtNs=50  pwmDtTicks=4  pwmReloadLogic=Full Cycle  pwmReloadFrequency=Every 1 PWM opportunity  pwmTriggeringSignal=Local force signal  pwmDutyCycleOutSim=off  pwmStartAfterInit=on  pwmShowAdvOpts=off  pwmPinA=PTA2: [PWM0_A3 | FlexPWM_0 Channel A Input/Output 3]  pwmPinB=None  pwmPolarityA=off  pwmPolarityB=off  pwmAInitialVal=0.25  pwmBInitialVal=0.25  pwmAShift=0  pwmBShift=0  trgReloadISR=off  trgVal0=off  trgVal1=off  trgVal2=off  trgVal3=off  trgVal4=off  trgVal5=off  trgReloadErrorISR=off  pwmPinFault=None  PwmFaultEnISR=off  pwmFaultEnA=off  pwmFaultEnB=off
  FlexPWM_Frequency_Update : mbd_mpc574x_ec_toolbox/Motor Control Blocks/FlexPWM Blocks/FlexPWM_Frequency_Update  Priority=1  pwmModule=0  pwmSubmodule0=off  pwmSubmodule1=off  pwmSubmodule2=off  pwmSubmodule3=on  pwmUnits=Hz
  wires:
  In1/1 -> FlexPWM_Frequency_Update/1
  In2/1 -> FlexPWM_Config/1

== system ZT_VehCtrl_18B_CAN/SigOut/GPIO /PWM_OUT/PWM Configuration and Frequency Update1 ==
  PWM A : Inport
  Fre A : Inport  Port=2
  PWM B : Inport  Port=3
  Fre B : Inport  Port=4
  Constant2 : Constant  Commented=on  Value=200
  Data Type Conversion : DataTypeConversion
  Data Type Conversion1 : DataTypeConversion
  Data Type Conversion2 : DataTypeConversion  Commented=on
  FlexPWM_Config : mbd_mpc574x_ec_toolbox/Motor Control Blocks/FlexPWM Blocks/FlexPWM_Config  Priority=1  pwmModule=0  pwmSubmodule=3  pwmMode=Center aligned PWM  pwmPair=Independent  pwmCompSource=PWM23  pwmCounterInit=Local sync (PWMX)  pwmClockSource=Peripheral clock  pwmUnits=Hz  pwmFrequency=200  pwmPeriod=25000  pwmPrescaler=Divide by 16  pwmDtUnits=Nanoseconds  pwmDtNs=50  pwmDtTicks=4  pwmReloadLogic=Full Cycle  pwmReloadFrequency=Every 1 PWM opportunity  pwmTriggeringSignal=Local force signal  pwmDutyCycleOutSim=off  pwmStartAfterInit=on  pwmShowAdvOpts=off  pwmPinA=PTD3: [PWM0_A3 | FlexPWM_0 Channel A Input/Output 3]  pwmPinB=PTD4: [PWM0_B3 | FlexPWM_0 Channel B Input/Output 3]  pwmPolarityA=off  pwmPolarityB=off  pwmAInitialVal=0.5  pwmBInitialVal=0.25  pwmAShift=0  pwmBShift=0  trgReloadISR=off  trgVal0=off  trgVal1=off  trgVal2=off  trgVal3=off  trgVal4=off  trgVal5=off  trgReloadErrorISR=off  pwmPinFault=None  PwmFaultEnISR=off  pwmFaultEnA=off  pwmFaultEnB=off
  FlexPWM_Frequency_Update : mbd_mpc574x_ec_toolbox/Motor Control Blocks/FlexPWM Blocks/FlexPWM_Frequency_Update  Priority=1  Commented=on  pwmModule=0  pwmSubmodule0=off  pwmSubmodule1=off  pwmSubmodule2=off  pwmSubmodule3=on  pwmUnits=Hz
  Terminator : Terminator
  Terminator1 : Terminator
  wires:
  Fre B/1 -> Terminator/1
  PWM A/1 -> Data Type Conversion/1
  Data Type Conversion/1 -> FlexPWM_Config/1
  PWM B/1 -> Data Type Conversion1/1
  Data Type Conversion1/1 -> FlexPWM_Config/2
  Fre A/1 -> Terminator1/1
  Constant2/1 -> Data Type Conversion2/1
  Data Type Conversion2/1 -> FlexPWM_Frequency_Update/1

== system ZT_VehCtrl_18B_CAN/SigOut/GPIO /PWM_OUT/PWM Configuration and Frequency Update4 ==
  PWM A : Inport
  Fre : Inport  Port=2
  Add : Sum  Inputs=+-
  Constant : Constant
  Constant1 : Constant  Commented=on  Value=200
  Data Type Conversion : DataTypeConversion
  Data Type Conversion1 : DataTypeConversion  Commented=on
  FlexPWM_Config : mbd_mpc574x_ec_toolbox/Motor Control Blocks/FlexPWM Blocks/FlexPWM_Config  Priority=1  pwmModule=0  pwmSubmodule=1  pwmMode=Center aligned PWM  pwmPair=Independent  pwmCompSource=PWM23  pwmCounterInit=Local sync (PWMX)  pwmClockSource=Peripheral clock  pwmUnits=Hz  pwmFrequency=200  pwmPeriod=25000  pwmPrescaler=Divide by 16  pwmDtUnits=Nanoseconds  pwmDtNs=50  pwmDtTicks=4  pwmReloadLogic=Full Cycle  pwmReloadFrequency=Every 1 PWM opportunity  pwmTriggeringSignal=Local force signal  pwmDutyCycleOutSim=off  pwmStartAfterInit=on  pwmShowAdvOpts=off  pwmPinA=PTC7: [PWM0_A1 | FlexPWM_0 Channel A Input/Output 1]  pwmPinB=None  pwmPolarityA=off  pwmPolarityB=off  pwmAInitialVal=0.25  pwmBInitialVal=0.25  pwmAShift=0  pwmBShift=0  trgReloadISR=off  trgVal0=off  trgVal1=off  trgVal2=off  trgVal3=off  trgVal4=off  trgVal5=off  trgReloadErrorISR=off  pwmPinFault=None  PwmFaultEnISR=off  pwmFaultEnA=off  pwmFaultEnB=off
  FlexPWM_Frequency_Update : mbd_mpc574x_ec_toolbox/Motor Control Blocks/FlexPWM Blocks/FlexPWM_Frequency_Update  Priority=1  Commented=on  pwmModule=0  pwmSubmodule0=off  pwmSubmodule1=on  pwmSubmodule2=off  pwmSubmodule3=off  pwmUnits=Hz
  Terminator : Terminator
  wires:
  PWM A/1 -> Add/2
  Add/1 -> Data Type Conversion/1
  Constant/1 -> Add/1
  Data Type Conversion/1 -> FlexPWM_Config/1
  Fre/1 -> Terminator/1
  Constant1/1 -> Data Type Conversion1/1
  Data Type Conversion1/1 -> FlexPWM_Frequency_Update/1

== system ZT_VehCtrl_18B_CAN/SigOut/GPIO /SPI0: LS09_14_15_16_1_2_11_4/LS_CTRL ==
  Enable : EnablePort
  Data Type Conversion3 : DataTypeConversion
  Data Type Conversion4 : DataTypeConversion
  Demux1 : Demux  Outputs=2
  If Action Subsystem1 : Subsystem  TreatAsAtomicUnit=on
  SPI_Master_Transfer_To1 : mbd_mpc574x_ec_toolbox/Communication Blocks/SPI Blocks/SPI_Master_Transfer  Priority=2  InstanceNumber=0  xfermode=Non blocking  timeout=50  spi_upd=on  WhichPCS=5
  Terminator : Terminator
  Terminator1 : Terminator
  Vector Concatenate1 : Concatenate
  wires:
  Vector Concatenate1/1 -> SPI_Master_Transfer_To1/1
  SPI_Master_Transfer_To1/1 -> Demux1/1
  Demux1/2 -> Data Type Conversion4/1
  Data Type Conversion3/1 -> Terminator/1
  Data Type Conversion4/1 -> Terminator1/1
  Demux1/1 -> Data Type Conversion3/1
  If Action Subsystem1/1(Out1) -> Vector Concatenate1/1
  If Action Subsystem1/2(Out2) -> Vector Concatenate1/2

== system ZT_VehCtrl_18B_CAN/SigOut/GPIO /SPI0: LS09_14_15_16_1_2_11_4/LS_CTRL1 ==
  Enable : EnablePort
  Data Type Conversion3 : DataTypeConversion
  Data Type Conversion4 : DataTypeConversion
  Demux1 : Demux  Outputs=2
  If Action Subsystem1 : Subsystem  TreatAsAtomicUnit=on
  SPI_Master_Transfer_To1 : mbd_mpc574x_ec_toolbox/Communication Blocks/SPI Blocks/SPI_Master_Transfer  Priority=2  InstanceNumber=0  xfermode=Non blocking  timeout=50  spi_upd=on  WhichPCS=1
  Terminator : Terminator
  Terminator1 : Terminator
  Vector Concatenate1 : Concatenate
  wires:
  Demux1/1 -> Data Type Conversion3/1
  Data Type Conversion4/1 -> Terminator1/1
  Data Type Conversion3/1 -> Terminator/1
  Demux1/2 -> Data Type Conversion4/1
  SPI_Master_Transfer_To1/1 -> Demux1/1
  Vector Concatenate1/1 -> SPI_Master_Transfer_To1/1
  If Action Subsystem1/2(Out2) -> Vector Concatenate1/2
  If Action Subsystem1/1(Out1) -> Vector Concatenate1/1

== system ZT_VehCtrl_18B_CAN/SigOut/GPIO /SPI3: LS03_06_07_08_10_12_13_17_18_19/Subsystem ==
  Enable : EnablePort
  Data Type Conversion : DataTypeConversion  OutDataTypeStr=uint8
  Data Type Conversion1 : DataTypeConversion  OutDataTypeStr=uint8
  Demux2 : Demux  Outputs=2
  SPI_Master_Transfer_To2 : mbd_mpc574x_ec_toolbox/Communication Blocks/SPI Blocks/SPI_Master_Transfer  Priority=2  InstanceNumber=3  xfermode=Non blocking  timeout=50  spi_upd=on  WhichPCS=3
  Terminator2 : Terminator
  Terminator3 : Terminator
  Vector Concatenate2 : Concatenate
  控制 : Subsystem  TreatAsAtomicUnit=on
  wires:
  Data Type Conversion1/1 -> Terminator3/1
  控制/2(Out2) -> Vector Concatenate2/2
  Demux2/1 -> Data Type Conversion/1
  Vector Concatenate2/1 -> SPI_Master_Transfer_To2/1
  Demux2/2 -> Data Type Conversion1/1
  Data Type Conversion/1 -> Terminator2/1
  控制/1(Out1) -> Vector Concatenate2/1
  SPI_Master_Transfer_To2/1 -> Demux2/1

== system ZT_VehCtrl_18B_CAN/SigIn/PWM/Subsystem/eTimer Configuration and Signal Measurements/Subsystem_capture ==
  In1 : Inport
  function : TriggerPort  TriggerType=function-call  VariantControl=Variant
  Terminator : Terminator
  eTimer_Arm_Capture : mbd_mpc574x_ec_toolbox/Motor Control Blocks/eTIMER Blocks/eTimer_Arm_Capture  etimerModule=0  etimerChannel=1  etimerArmAction=Stop
  eTimer_Capture : mbd_mpc574x_ec_toolbox/Motor Control Blocks/eTIMER Blocks/eTimer_Capture  etimerModule=0  etimerChannel=1
  Out1 : Outport  OutDataTypeStr=uint16
  Out2 : Outport  Port=2  OutDataTypeStr=uint16
  Out3 : Outport  Port=3  OutDataTypeStr=uint16
  Out4 : Outport  Port=4  OutDataTypeStr=uint16
  wires:
  eTimer_Capture/1 -> Out1/1
  eTimer_Capture/4 -> Out4/1
  eTimer_Capture/3 -> Out3/1
  eTimer_Capture/2 -> Out2/1
  In1/1 -> Terminator/1

== system ZT_VehCtrl_18B_CAN/SigOut/GPIO /SPI0: LS09_14_15_16_1_2_11_4/LS_CTRL/If Action Subsystem1 ==
  Add : Sum  Inputs=++++
  Constant1 : Constant  Value=128  OutDataTypeStr=uint8
  Constant2 : Constant  Value=64  OutDataTypeStr=uint8
  Constant3 : Constant  Value=32  OutDataTypeStr=uint8
  Constant4 : Constant  Value=16  OutDataTypeStr=uint8
  Constant5 : Constant  Value=8  OutDataTypeStr=uint8
  Constant6 : Constant  Value=4  OutDataTypeStr=uint8
  Constant7 : Constant  Value=2  OutDataTypeStr=uint8
  Constant8 : Constant  OutDataTypeStr=uint8
  Constant9 : Constant  Value=128  OutDataTypeStr=uint8
  Data Store Read : DataStoreRead  DataStoreName=LS004
  Data Store Read4 : DataStoreRead  DataStoreName=LS011
  Data Store Read5 : DataStoreRead  DataStoreName=LS001
  Data Store Read6 : DataStoreRead  DataStoreName=LS002
  Data Type Conversion : DataTypeConversion
  Data Type Conversion1 : DataTypeConversion
  Switch{,1..3} (4 alike) : Switch  Criteria=u2 > Threshold
  Out1 : Outport
  Out2 : Outport  Port=2
  wires:
  Constant2/1 -> Switch/3
  Constant1/1 -> Switch/1
  Add/1 -> Data Type Conversion1/1
  Data Store Read6/1 -> Switch/2
  Constant7/1 -> Switch3/1
  Switch1/1 -> Add/2
  Constant5/1 -> Switch2/1
  Switch/1 -> Add/1
  Constant4/1 -> Switch1/3
  Data Store Read/1 -> Switch3/2
  Switch2/1 -> Add/3
  Data Store Read4/1 -> Switch2/2
  Switch3/1 -> Add/4
  Constant3/1 -> Switch1/1
  Data Store Read5/1 -> Switch1/2
  Constant8/1 -> Switch3/3
  Constant9/1 -> Data Type Conversion/1
  Constant6/1 -> Switch2/3
  Data Type Conversion/1 -> Out1/1
  Data Type Conversion1/1 -> Out2/1

== system ZT_VehCtrl_18B_CAN/SigOut/GPIO /SPI0: LS09_14_15_16_1_2_11_4/LS_CTRL1/If Action Subsystem1 ==
  Add : Sum  Inputs=++++
  Constant1 : Constant  Value=128  OutDataTypeStr=uint8
  Constant2 : Constant  Value=64  OutDataTypeStr=uint8
  Constant3 : Constant  Value=32  OutDataTypeStr=uint8
  Constant4 : Constant  Value=16  OutDataTypeStr=uint8
  Constant5 : Constant  Value=8  OutDataTypeStr=uint8
  Constant6 : Constant  Value=4  OutDataTypeStr=uint8
  Constant7 : Constant  Value=2  OutDataTypeStr=uint8
  Constant8 : Constant  OutDataTypeStr=uint8
  Constant9 : Constant  Value=128  OutDataTypeStr=uint8
  Data Store Read : DataStoreRead  DataStoreName=LS014
  Data Store Read4 : DataStoreRead  DataStoreName=LS015
  Data Store Read5 : DataStoreRead  DataStoreName=LS009
  Data Store Read6 : DataStoreRead  DataStoreName=LS016
  Data Type Conversion : DataTypeConversion
  Data Type Conversion1 : DataTypeConversion
  Switch{,1..3} (4 alike) : Switch  Criteria=u2 > Threshold
  Out1 : Outport
  Out2 : Outport  Port=2
  wires:
  Data Type Conversion1/1 -> Out2/1
  Data Type Conversion/1 -> Out1/1
  Constant6/1 -> Switch2/3
  Constant9/1 -> Data Type Conversion/1
  Constant8/1 -> Switch3/3
  Data Store Read5/1 -> Switch1/2
  Constant3/1 -> Switch1/1
  Switch3/1 -> Add/4
  Data Store Read4/1 -> Switch2/2
  Switch2/1 -> Add/3
  Data Store Read/1 -> Switch3/2
  Constant4/1 -> Switch1/3
  Switch/1 -> Add/1
  Constant5/1 -> Switch2/1
  Switch1/1 -> Add/2
  Constant7/1 -> Switch3/1
  Data Store Read6/1 -> Switch/2
  Add/1 -> Data Type Conversion1/1
  Constant1/1 -> Switch/1
  Constant2/1 -> Switch/3
